simulink model "ATOM_parking_chain"  (R2026a)
settings: Solver=ode4  StopTime=100  FixedStep=0.01
StopFcn:
  | % Put every new figure in the same MATLAB Figures window as a docked tab.
  | set(groot, 'defaultFigureWindowStyle', 'docked');
  | 
  | if exist('costmap_active', 'var') && ...
  |         exist('vehicle', 'var') && ...
  |         exist('parking_path', 'var') && ...
  |         ~isempty(parking_path)
  | 
  |     plotPlan(costmap_active, vehicle, parking_path);
  | 
  | else
  | 
  |     warning('No valid parking path is available for plotting.');
  | 
  | end
  | 
  | PlotControllerReferences( ...
  |     out.controller_reference_log);
  | 
  | PlotControllerTracking( ...
  |     out.controller_tracking_log);
undefined symbols (not defined in the file): lateral, longitudinal, stanley, vehicle
(part 2 of 11)

== system ATOM_parking_chain/time_parameterization2 ==
  trajectory_in : Inport
  steer_rate_limit : Inport  Port=2
  Time parameterization : MATLAB Function  TreatAsAtomicUnit=on
  To Workspace : ToWorkspace  VariableName=time_parameterized_reference_log  SaveFormat=Timeseries  SampleTime=-1
  reference_out : Outport
  wires:
  trajectory_in/1 -> Time parameterization/1(trajectory_in)
  Time parameterization/1(reference_out) -> To Workspace/1, reference_out/1
  steer_rate_limit/1 -> Time parameterization/2(steer_rate_limit)

== system ATOM_parking_chain/Parking Scenario/Costmap generation: complex parking situation ==
  From Workspace1 : FromWorkspace  VariableName=veh
  MATLAB Function : MATLAB Function  TreatAsAtomicUnit=on
  costmap : Outport
  start_pose : Outport  Port=2
  goal_pose : Outport  Port=3
  wires:
  MATLAB Function/1(costmap) -> costmap/1
  From Workspace1/1 -> MATLAB Function/1(veh)
  MATLAB Function/2(start_pose) -> start_pose/1
  MATLAB Function/3(goal_pose) -> goal_pose/1

== system ATOM_parking_chain/Parking Scenario/Costmap generation: corridor occupancy grid ==
  From Workspace1 : FromWorkspace  VariableName=veh
  MATLAB Function : MATLAB Function  TreatAsAtomicUnit=on
  costmap : Outport
  start_pose : Outport  Port=2
  goal_pose : Outport  Port=3
  wires:
  MATLAB Function/1(costmap) -> costmap/1
  From Workspace1/1 -> MATLAB Function/1(veh)
  MATLAB Function/3(goal_pose) -> goal_pose/1
  MATLAB Function/2(start_pose) -> start_pose/1

== system ATOM_parking_chain/Parking Scenario/Costmap generation: empty occupancy grid ==
  From Workspace1 : FromWorkspace  VariableName=veh
  MATLAB Function : MATLAB Function  TreatAsAtomicUnit=on
  costmap : Outport
  start_pose : Outport  Port=2
  goal_pose : Outport  Port=3
  wires:
  MATLAB Function/1(costmap) -> costmap/1
  From Workspace1/1 -> MATLAB Function/1(veh)
  MATLAB Function/2(start_pose) -> start_pose/1
  MATLAB Function/3(goal_pose) -> goal_pose/1

== system ATOM_parking_chain/Parking Scenario/Costmap generation: obstacle ==
  From Workspace1 : FromWorkspace  VariableName=veh
  MATLAB Function : MATLAB Function  TreatAsAtomicUnit=on
  costmap : Outport
  start_pose : Outport  Port=2
  goal_pose : Outport  Port=3
  wires:
  MATLAB Function/1(costmap) -> costmap/1
  From Workspace1/1 -> MATLAB Function/1(veh)
  MATLAB Function/2(start_pose) -> start_pose/1
  MATLAB Function/3(goal_pose) -> goal_pose/1

== system ATOM_parking_chain/Parking Scenario/Costmap generation: obstacle1 ==
  From Workspace1 : FromWorkspace  VariableName=veh
  MATLAB Function : MATLAB Function  TreatAsAtomicUnit=on
  costmap : Outport
  start_pose : Outport  Port=2
  goal_pose : Outport  Port=3
  wires:
  MATLAB Function/1(costmap) -> costmap/1
  From Workspace1/1 -> MATLAB Function/1(veh)
  MATLAB Function/2(start_pose) -> start_pose/1
  MATLAB Function/3(goal_pose) -> goal_pose/1

== system ATOM_parking_chain/Parking Scenario/Costmap generation: obstacle2 ==
  From Workspace1 : FromWorkspace  VariableName=veh
  MATLAB Function : MATLAB Function  TreatAsAtomicUnit=on
  costmap : Outport
  start_pose : Outport  Port=2
  goal_pose : Outport  Port=3
  wires:
  MATLAB Function/1(costmap) -> costmap/1
  From Workspace1/1 -> MATLAB Function/1(veh)
  MATLAB Function/2(start_pose) -> start_pose/1
  MATLAB Function/3(goal_pose) -> goal_pose/1

== system ATOM_parking_chain/Parking Scenario/Costmap generation: parking scenario beside a lane ==
  From Workspace1 : FromWorkspace  VariableName=veh
  MATLAB Function : MATLAB Function  TreatAsAtomicUnit=on
  costmap : Outport
  start_pose : Outport  Port=2
  goal_pose : Outport  Port=3
  wires:
  MATLAB Function/1(costmap) -> costmap/1
  From Workspace1/1 -> MATLAB Function/1(veh)
  MATLAB Function/2(start_pose) -> start_pose/1
  MATLAB Function/3(goal_pose) -> goal_pose/1

== system ATOM_parking_chain/Parking Scenario/Costmap generation: perpendicular lot ==
  From Workspace1 : FromWorkspace  VariableName=veh
  Perpendicular Parking : MATLAB Function  TreatAsAtomicUnit=on
  costmap : Outport
  start_pose : Outport  Port=2
  goal_pose : Outport  Port=3
  wires:
  Perpendicular Parking/1(costmap) -> costmap/1
  From Workspace1/1 -> Perpendicular Parking/1(veh)
  Perpendicular Parking/2(start_pose) -> start_pose/1
  Perpendicular Parking/3(goal_pose) -> goal_pose/1

== system ATOM_parking_chain/Parking Scenario/freespace_planner ==
  costmap : Inport
  veh : Inport  Port=2
  goal_pose : Inport  Port=3
  start_pose : Inport  Port=4
  segment_request : Inport  Port=5
  Bus Creator3 : BusCreator  Inputs=3  OutDataTypeStr=Bus: PointBusN
  Bus Creator4 : BusCreator  Inputs=4  OutDataTypeStr=Bus: QuaternionBusN
  Bus Creator5 : BusCreator  Inputs=2  OutDataTypeStr=Bus: PoseBusN
      settings: InheritFromInputs=off
  Bus Creator6 : BusCreator  Inputs=7  OutDataTypeStr=Bus: TrajectoryDataBus
      settings: InheritFromInputs=off
  freespacePlanner : MATLAB Function  TreatAsAtomicUnit=on
  traj : Outport
  segment_count : Outport  Port=2
  wires:
  Bus Creator6/1 -> traj/1
  Bus Creator3/1 -> Bus Creator5/1
  freespacePlanner/13(rear_wheel_angle_rad) -> Bus Creator6/7
  Bus Creator5/1 -> Bus Creator6/1
  freespacePlanner/8(longitudinal_velocity_mps) -> Bus Creator6/2
  freespacePlanner/3(z) -> Bus Creator3/3
  freespacePlanner/4(qx) -> Bus Creator4/1
  freespacePlanner/9(lateral_velocity_mps) -> Bus Creator6/3
  freespacePlanner/10(acceleration_mps2) -> Bus Creator6/4
  freespacePlanner/5(qy) -> Bus Creator4/2
  freespacePlanner/1(x) -> Bus Creator3/1
  freespacePlanner/2(y) -> Bus Creator3/2
  freespacePlanner/7(qw) -> Bus Creator4/4
  freespacePlanner/6(qz) -> Bus Creator4/3
  freespacePlanner/12(front_wheel_angle_rad) -> Bus Creator6/6
  Bus Creator4/1 -> Bus Creator5/2
  freespacePlanner/11(heading_rate_rps) -> Bus Creator6/5
  costmap/1 -> freespacePlanner/4(costmap)
  start_pose/1 -> freespacePlanner/1(start_pose)
  goal_pose/1 -> freespacePlanner/2(goal_pose)
  veh/1 -> freespacePlanner/3(veh)
  segment_request/1 -> freespacePlanner/5(segment_request)
  freespacePlanner/14(segment_count) -> segment_count/1

== system ATOM_parking_chain/Parking Scenario1/Costmap generation: complex parking situation ==
  From Workspace1 : FromWorkspace  VariableName=veh
  MATLAB Function : MATLAB Function  TreatAsAtomicUnit=on
  costmap : Outport
  start_pose : Outport  Port=2
  goal_pose : Outport  Port=3
  wires:
  MATLAB Function/1(costmap) -> costmap/1
  From Workspace1/1 -> MATLAB Function/1(veh)
  MATLAB Function/2(start_pose) -> start_pose/1
  MATLAB Function/3(goal_pose) -> goal_pose/1

== system ATOM_parking_chain/Parking Scenario1/Costmap generation: corridor occupancy grid ==
  From Workspace1 : FromWorkspace  VariableName=veh
  MATLAB Function : MATLAB Function  TreatAsAtomicUnit=on
  costmap : Outport
  start_pose : Outport  Port=2
  goal_pose : Outport  Port=3
  wires:
  MATLAB Function/1(costmap) -> costmap/1
  From Workspace1/1 -> MATLAB Function/1(veh)
  MATLAB Function/3(goal_pose) -> goal_pose/1
  MATLAB Function/2(start_pose) -> start_pose/1

== system ATOM_parking_chain/Parking Scenario1/Costmap generation: empty occupancy grid ==
  From Workspace1 : FromWorkspace  VariableName=veh
  MATLAB Function : MATLAB Function  TreatAsAtomicUnit=on
  costmap : Outport
  start_pose : Outport  Port=2
  goal_pose : Outport  Port=3
  wires:
  MATLAB Function/1(costmap) -> costmap/1
  From Workspace1/1 -> MATLAB Function/1(veh)
  MATLAB Function/2(start_pose) -> start_pose/1
  MATLAB Function/3(goal_pose) -> goal_pose/1

== system ATOM_parking_chain/Parking Scenario1/Costmap generation: obstacle ==
  From Workspace1 : FromWorkspace  VariableName=veh
  MATLAB Function : MATLAB Function  TreatAsAtomicUnit=on
  costmap : Outport
  start_pose : Outport  Port=2
  goal_pose : Outport  Port=3
  wires:
  MATLAB Function/1(costmap) -> costmap/1
  From Workspace1/1 -> MATLAB Function/1(veh)
  MATLAB Function/2(start_pose) -> start_pose/1
  MATLAB Function/3(goal_pose) -> goal_pose/1

== system ATOM_parking_chain/Parking Scenario1/Costmap generation: obstacle1 ==
  From Workspace1 : FromWorkspace  VariableName=veh
  MATLAB Function : MATLAB Function  TreatAsAtomicUnit=on
  costmap : Outport
  start_pose : Outport  Port=2
  goal_pose : Outport  Port=3
  wires:
  MATLAB Function/1(costmap) -> costmap/1
  From Workspace1/1 -> MATLAB Function/1(veh)
  MATLAB Function/2(start_pose) -> start_pose/1
  MATLAB Function/3(goal_pose) -> goal_pose/1

== system ATOM_parking_chain/Parking Scenario1/Costmap generation: obstacle2 ==
  From Workspace1 : FromWorkspace  VariableName=veh
  MATLAB Function : MATLAB Function  TreatAsAtomicUnit=on
  costmap : Outport
  start_pose : Outport  Port=2
  goal_pose : Outport  Port=3
  wires:
  MATLAB Function/1(costmap) -> costmap/1
  From Workspace1/1 -> MATLAB Function/1(veh)
  MATLAB Function/2(start_pose) -> start_pose/1
  MATLAB Function/3(goal_pose) -> goal_pose/1

== system ATOM_parking_chain/Parking Scenario1/Costmap generation: parking scenario beside a lane ==
  From Workspace1 : FromWorkspace  VariableName=veh
  MATLAB Function : MATLAB Function  TreatAsAtomicUnit=on
  costmap : Outport
  start_pose : Outport  Port=2
  goal_pose : Outport  Port=3
  wires:
  MATLAB Function/1(costmap) -> costmap/1
  From Workspace1/1 -> MATLAB Function/1(veh)
  MATLAB Function/2(start_pose) -> start_pose/1
  MATLAB Function/3(goal_pose) -> goal_pose/1

== system ATOM_parking_chain/Parking Scenario1/Costmap generation: perpendicular lot ==
  From Workspace1 : FromWorkspace  VariableName=veh
  Perpendicular Parking : MATLAB Function  TreatAsAtomicUnit=on
  costmap : Outport
  start_pose : Outport  Port=2
  goal_pose : Outport  Port=3
  wires:
  Perpendicular Parking/1(costmap) -> costmap/1
  From Workspace1/1 -> Perpendicular Parking/1(veh)
  Perpendicular Parking/2(start_pose) -> start_pose/1
  Perpendicular Parking/3(goal_pose) -> goal_pose/1

== system ATOM_parking_chain/Parking Scenario1/freespace_planner ==
  costmap : Inport
  veh : Inport  Port=2
  goal_pose : Inport  Port=3
  start_pose : Inport  Port=4
  segment_request : Inport  Port=5
  Bus Creator3 : BusCreator  Inputs=3  OutDataTypeStr=Bus: PointBusN
  Bus Creator4 : BusCreator  Inputs=4  OutDataTypeStr=Bus: QuaternionBusN
  Bus Creator5 : BusCreator  Inputs=2  OutDataTypeStr=Bus: PoseBusN
      settings: InheritFromInputs=off
  Bus Creator6 : BusCreator  Inputs=7  OutDataTypeStr=Bus: TrajectoryDataBus
      settings: InheritFromInputs=off
  freespacePlanner : MATLAB Function  TreatAsAtomicUnit=on
  traj : Outport
  segment_count : Outport  Port=2
  wires:
  Bus Creator6/1 -> traj/1
  Bus Creator3/1 -> Bus Creator5/1
  freespacePlanner/13(rear_wheel_angle_rad) -> Bus Creator6/7
  Bus Creator5/1 -> Bus Creator6/1
  freespacePlanner/8(longitudinal_velocity_mps) -> Bus Creator6/2
  freespacePlanner/3(z) -> Bus Creator3/3
  freespacePlanner/4(qx) -> Bus Creator4/1
  freespacePlanner/9(lateral_velocity_mps) -> Bus Creator6/3
  freespacePlanner/10(acceleration_mps2) -> Bus Creator6/4
  freespacePlanner/5(qy) -> Bus Creator4/2
  freespacePlanner/1(x) -> Bus Creator3/1
  freespacePlanner/2(y) -> Bus Creator3/2
  freespacePlanner/7(qw) -> Bus Creator4/4
  freespacePlanner/6(qz) -> Bus Creator4/3
  freespacePlanner/12(front_wheel_angle_rad) -> Bus Creator6/6
  Bus Creator4/1 -> Bus Creator5/2
  freespacePlanner/11(heading_rate_rps) -> Bus Creator6/5
  costmap/1 -> freespacePlanner/4(costmap)
  start_pose/1 -> freespacePlanner/1(start_pose)
  goal_pose/1 -> freespacePlanner/2(goal_pose)
  veh/1 -> freespacePlanner/3(veh)
  segment_request/1 -> freespacePlanner/5(segment_request)
  freespacePlanner/14(segment_count) -> segment_count/1

== system ATOM_parking_chain/Parking Scenario2/Costmap generation: complex parking situation ==
  From Workspace1 : FromWorkspace  VariableName=veh
  MATLAB Function : MATLAB Function  TreatAsAtomicUnit=on
  costmap : Outport
  start_pose : Outport  Port=2
  goal_pose : Outport  Port=3
  wires:
  MATLAB Function/1(costmap) -> costmap/1
  From Workspace1/1 -> MATLAB Function/1(veh)
  MATLAB Function/2(start_pose) -> start_pose/1
  MATLAB Function/3(goal_pose) -> goal_pose/1

== system ATOM_parking_chain/Parking Scenario2/Costmap generation: corridor occupancy grid ==
  From Workspace1 : FromWorkspace  VariableName=veh
  MATLAB Function : MATLAB Function  TreatAsAtomicUnit=on
  costmap : Outport
  start_pose : Outport  Port=2
  goal_pose : Outport  Port=3
  wires:
  MATLAB Function/1(costmap) -> costmap/1
  From Workspace1/1 -> MATLAB Function/1(veh)
  MATLAB Function/3(goal_pose) -> goal_pose/1
  MATLAB Function/2(start_pose) -> start_pose/1

== system ATOM_parking_chain/Parking Scenario2/Costmap generation: empty occupancy grid ==
  From Workspace1 : FromWorkspace  VariableName=veh
  MATLAB Function : MATLAB Function  TreatAsAtomicUnit=on
  costmap : Outport
  start_pose : Outport  Port=2
  goal_pose : Outport  Port=3
  wires:
  MATLAB Function/1(costmap) -> costmap/1
  From Workspace1/1 -> MATLAB Function/1(veh)
  MATLAB Function/2(start_pose) -> start_pose/1
  MATLAB Function/3(goal_pose) -> goal_pose/1

== system ATOM_parking_chain/Parking Scenario2/Costmap generation: obstacle ==
  From Workspace1 : FromWorkspace  VariableName=veh
  MATLAB Function : MATLAB Function  TreatAsAtomicUnit=on
  costmap : Outport
  start_pose : Outport  Port=2
  goal_pose : Outport  Port=3
  wires:
  MATLAB Function/1(costmap) -> costmap/1
  From Workspace1/1 -> MATLAB Function/1(veh)
  MATLAB Function/2(start_pose) -> start_pose/1
  MATLAB Function/3(goal_pose) -> goal_pose/1

== system ATOM_parking_chain/Parking Scenario2/Costmap generation: obstacle1 ==
  From Workspace1 : FromWorkspace  VariableName=veh
  MATLAB Function : MATLAB Function  TreatAsAtomicUnit=on
  costmap : Outport
  start_pose : Outport  Port=2
  goal_pose : Outport  Port=3
  wires:
  MATLAB Function/1(costmap) -> costmap/1
  From Workspace1/1 -> MATLAB Function/1(veh)
  MATLAB Function/2(start_pose) -> start_pose/1
  MATLAB Function/3(goal_pose) -> goal_pose/1

== system ATOM_parking_chain/Parking Scenario2/Costmap generation: obstacle2 ==
  From Workspace1 : FromWorkspace  VariableName=veh
  MATLAB Function : MATLAB Function  TreatAsAtomicUnit=on
  costmap : Outport
  start_pose : Outport  Port=2
  goal_pose : Outport  Port=3
  wires:
  MATLAB Function/1(costmap) -> costmap/1
  From Workspace1/1 -> MATLAB Function/1(veh)
  MATLAB Function/2(start_pose) -> start_pose/1
  MATLAB Function/3(goal_pose) -> goal_pose/1

== system ATOM_parking_chain/Parking Scenario2/Costmap generation: parking scenario beside a lane ==
  From Workspace1 : FromWorkspace  VariableName=veh
  MATLAB Function : MATLAB Function  TreatAsAtomicUnit=on
  costmap : Outport
  start_pose : Outport  Port=2
  goal_pose : Outport  Port=3
  wires:
  MATLAB Function/1(costmap) -> costmap/1
  From Workspace1/1 -> MATLAB Function/1(veh)
  MATLAB Function/2(start_pose) -> start_pose/1
  MATLAB Function/3(goal_pose) -> goal_pose/1

== system ATOM_parking_chain/Parking Scenario2/Costmap generation: perpendicular lot ==
  From Workspace1 : FromWorkspace  VariableName=veh
  Perpendicular Parking : MATLAB Function  TreatAsAtomicUnit=on
  costmap : Outport
  start_pose : Outport  Port=2
  goal_pose : Outport  Port=3
  wires:
  Perpendicular Parking/1(costmap) -> costmap/1
  From Workspace1/1 -> Perpendicular Parking/1(veh)
  Perpendicular Parking/2(start_pose) -> start_pose/1
  Perpendicular Parking/3(goal_pose) -> goal_pose/1

== system ATOM_parking_chain/Parking Scenario2/freespace_planner ==
  costmap : Inport
  veh : Inport  Port=2
  goal_pose : Inport  Port=3
  start_pose : Inport  Port=4
  segment_request : Inport  Port=5
  Bus Creator3 : BusCreator  Inputs=3  OutDataTypeStr=Bus: PointBusN
  Bus Creator4 : BusCreator  Inputs=4  OutDataTypeStr=Bus: QuaternionBusN
  Bus Creator5 : BusCreator  Inputs=2  OutDataTypeStr=Bus: PoseBusN
      settings: InheritFromInputs=off
  Bus Creator6 : BusCreator  Inputs=7  OutDataTypeStr=Bus: TrajectoryDataBus
      settings: InheritFromInputs=off
  freespacePlanner : MATLAB Function  TreatAsAtomicUnit=on
  traj : Outport
  segment_count : Outport  Port=2
  wires:
  Bus Creator6/1 -> traj/1
  Bus Creator3/1 -> Bus Creator5/1
  freespacePlanner/13(rear_wheel_angle_rad) -> Bus Creator6/7
  Bus Creator5/1 -> Bus Creator6/1
  freespacePlanner/8(longitudinal_velocity_mps) -> Bus Creator6/2
  freespacePlanner/3(z) -> Bus Creator3/3
  freespacePlanner/4(qx) -> Bus Creator4/1
  freespacePlanner/9(lateral_velocity_mps) -> Bus Creator6/3
  freespacePlanner/10(acceleration_mps2) -> Bus Creator6/4
  freespacePlanner/5(qy) -> Bus Creator4/2
  freespacePlanner/1(x) -> Bus Creator3/1
  freespacePlanner/2(y) -> Bus Creator3/2
  freespacePlanner/7(qw) -> Bus Creator4/4
  freespacePlanner/6(qz) -> Bus Creator4/3
  freespacePlanner/12(front_wheel_angle_rad) -> Bus Creator6/6
  Bus Creator4/1 -> Bus Creator5/2
  freespacePlanner/11(heading_rate_rps) -> Bus Creator6/5
  costmap/1 -> freespacePlanner/4(costmap)
  start_pose/1 -> freespacePlanner/1(start_pose)
  goal_pose/1 -> freespacePlanner/2(goal_pose)
  veh/1 -> freespacePlanner/3(veh)
  segment_request/1 -> freespacePlanner/5(segment_request)
  freespacePlanner/14(segment_count) -> segment_count/1

== system ATOM_parking_chain/Plot vehicle1/SetStanleyTrajectory ==
  ref_traj : Inport
  ego_pose : Inport  Port=2
  Constant1 : Constant  Value=stanley.traj_resample_dist
  Resample Trajectory : MATLAB Function  TreatAsAtomicUnit=on
  calcLongOffsetToSegment : MATLAB Function  TreatAsAtomicUnit=on
  default : Constant  Value=3
  default1 : Constant  Value=pi/2
  findFirstNearestSegmentIndexWithSoftConstraints : MATLAB Function  TreatAsAtomicUnit=on
  trajectory_out : Outport
  wires:
  ref_traj/1 -> Resample Trajectory/1(trajectory_in), calcLongOffsetToSegment/3(trajectory), findFirstNearestSegmentIndexWithSoftConstraints/1(trajectory)
  Constant1/1 -> Resample Trajectory/2(resample_interval_dist)
  calcLongOffsetToSegment/1(ego_offset_to_segment) -> Resample Trajectory/4(ego_offset_to_segment)
  ego_pose/1 -> findFirstNearestSegmentIndexWithSoftConstraints/4(pose), calcLongOffsetToSegment/2(ego_pose)
  findFirstNearestSegmentIndexWithSoftConstraints/1(nearest_seg_idx) -> calcLongOffsetToSegment/1(seg_idx), Resample Trajectory/3(nearest_seg_idx)
  default/1 -> findFirstNearestSegmentIndexWithSoftConstraints/2(dist_threshold)
  default1/1 -> findFirstNearestSegmentIndexWithSoftConstraints/3(yaw_threshold)
  Resample Trajectory/1(trajectory_out) -> trajectory_out/1

== system ATOM_parking_chain/Plot vehicle2/SetStanleyTrajectory ==
  ref_traj : Inport
  ego_pose : Inport  Port=2
  Constant1 : Constant  Value=stanley.traj_resample_dist
  Resample Trajectory : MATLAB Function  TreatAsAtomicUnit=on
  calcLongOffsetToSegment : MATLAB Function  TreatAsAtomicUnit=on
  default : Constant  Value=3
  default1 : Constant  Value=pi/2
  findFirstNearestSegmentIndexWithSoftConstraints : MATLAB Function  TreatAsAtomicUnit=on
  trajectory_out : Outport
  wires:
  ref_traj/1 -> Resample Trajectory/1(trajectory_in), calcLongOffsetToSegment/3(trajectory), findFirstNearestSegmentIndexWithSoftConstraints/1(trajectory)
  Constant1/1 -> Resample Trajectory/2(resample_interval_dist)
  calcLongOffsetToSegment/1(ego_offset_to_segment) -> Resample Trajectory/4(ego_offset_to_segment)
  ego_pose/1 -> findFirstNearestSegmentIndexWithSoftConstraints/4(pose), calcLongOffsetToSegment/2(ego_pose)
  findFirstNearestSegmentIndexWithSoftConstraints/1(nearest_seg_idx) -> calcLongOffsetToSegment/1(seg_idx), Resample Trajectory/3(nearest_seg_idx)
  default/1 -> findFirstNearestSegmentIndexWithSoftConstraints/2(dist_threshold)
  default1/1 -> findFirstNearestSegmentIndexWithSoftConstraints/3(yaw_threshold)
  Resample Trajectory/1(trajectory_out) -> trajectory_out/1

== system ATOM_parking_chain/Plot vehicle3/SetStanleyTrajectory ==
  ref_traj : Inport
  ego_pose : Inport  Port=2
  Constant1 : Constant  Value=stanley.traj_resample_dist
  Resample Trajectory : MATLAB Function  TreatAsAtomicUnit=on
  calcLongOffsetToSegment : MATLAB Function  TreatAsAtomicUnit=on
  default : Constant  Value=3
  default1 : Constant  Value=pi/2
  findFirstNearestSegmentIndexWithSoftConstraints : MATLAB Function  TreatAsAtomicUnit=on
  trajectory_out : Outport
  wires:
  ref_traj/1 -> Resample Trajectory/1(trajectory_in), calcLongOffsetToSegment/3(trajectory), findFirstNearestSegmentIndexWithSoftConstraints/1(trajectory)
  Constant1/1 -> Resample Trajectory/2(resample_interval_dist)
  calcLongOffsetToSegment/1(ego_offset_to_segment) -> Resample Trajectory/4(ego_offset_to_segment)
  ego_pose/1 -> findFirstNearestSegmentIndexWithSoftConstraints/4(pose), calcLongOffsetToSegment/2(ego_pose)
  findFirstNearestSegmentIndexWithSoftConstraints/1(nearest_seg_idx) -> calcLongOffsetToSegment/1(seg_idx), Resample Trajectory/3(nearest_seg_idx)
  default/1 -> findFirstNearestSegmentIndexWithSoftConstraints/2(dist_threshold)
  default1/1 -> findFirstNearestSegmentIndexWithSoftConstraints/3(yaw_threshold)
  Resample Trajectory/1(trajectory_out) -> trajectory_out/1

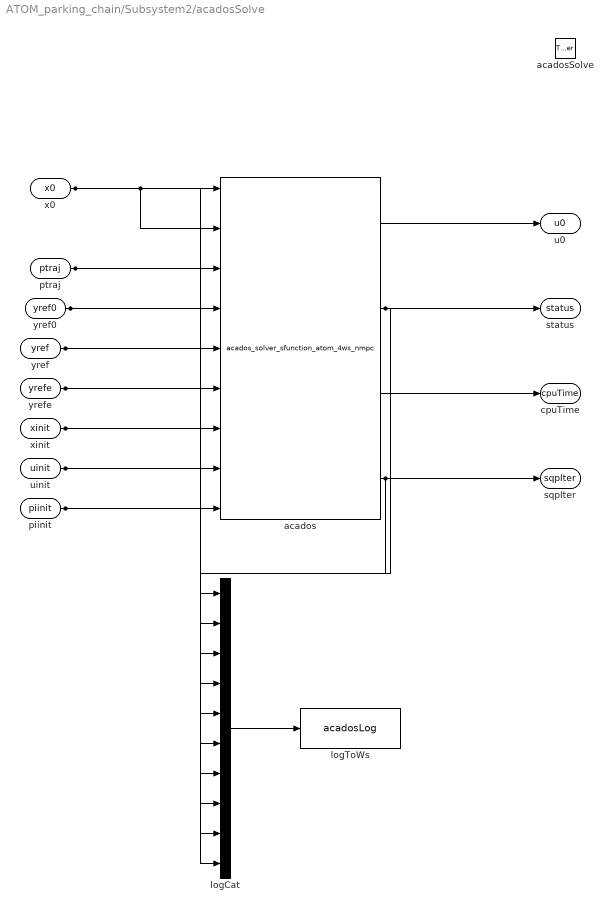
== system ATOM_parking_chain/Subsystem2/acadosSolve ==
  acadosSolve : TriggerPort  TriggerType=function-call  IsSimulinkFunction=on  FunctionName=acadosSolve  FunctionVisibility=scoped  VariantControl=(inherit)
  acados : S-Function  FunctionName=acados_solver_sfunction_atom_4ws_nmpc  SFunctionDeploymentMode=off  EnableBusSupport=off
  logCat : Concatenate  NumInputs=10
  logToWs : ToWorkspace  VariableName=acadosLog  SaveFormat=Structure With Time  SampleTime=-1
  x0 : ArgIn  DisableCoverage=on  PortDimensions=[9 1]  ArgumentName=x0
  ptraj : ArgIn  Port=2  PortDimensions=[272 1]  ArgumentName=ptraj
  yref0 : ArgIn  Port=3  PortDimensions=[7 1]  ArgumentName=yref0
  yref : ArgIn  Port=4  PortDimensions=[98 1]  ArgumentName=yref
  yrefe : ArgIn  Port=5  PortDimensions=[5 1]  ArgumentName=yrefe
  xinit : ArgIn  Port=6  PortDimensions=[144 1]  ArgumentName=xinit
  uinit : ArgIn  Port=7  PortDimensions=[30 1]  ArgumentName=uinit
  piinit : ArgIn  Port=8  PortDimensions=[135 1]  ArgumentName=piinit
  u0 : ArgOut  DisableCoverage=on  PortDimensions=[2 1]  ArgumentName=u0
  status : ArgOut  Port=2  ArgumentName=status
  cpuTime : ArgOut  Port=3  ArgumentName=cpuTime
  sqpIter : ArgOut  Port=4  ArgumentName=sqpIter
  wires:
  x0/1 -> acados/1, acados/2, logCat/1
  ptraj/1 -> acados/3, logCat/2
  yref0/1 -> acados/4, logCat/3
  yref/1 -> acados/5, logCat/4
  yrefe/1 -> acados/6, logCat/5
  xinit/1 -> acados/7, logCat/6
  uinit/1 -> acados/8, logCat/7
  piinit/1 -> acados/9, logCat/8
  acados/1 -> u0/1
  acados/2 -> status/1, logCat/9
  acados/3 -> cpuTime/1
  acados/4 -> sqpIter/1, logCat/10
  logCat/1 -> logToWs/1

== system ATOM_parking_chain/Vehicle_Model/Vehicle Dynamics ==
  command : Inport
  rear_steer_command : Inport  Port=2
  From Workspace : FromWorkspace  VariableName=veh
  MATLAB Function : MATLAB Function  TreatAsAtomicUnit=on
  state integrator : Subsystem
  IntState : Outport
  wires:
  command/1 -> MATLAB Function/2(command)
  MATLAB Function/1(d_state) -> state integrator/1(d_state)  "d_state"
  state integrator/1(state) -> MATLAB Function/1(state), IntState/1
  From Workspace/1 -> MATLAB Function/3(veh)
  rear_steer_command/1 -> MATLAB Function/4(rear_steering_command)

== system ATOM_parking_chain/Vehicle_Model/Vehicle internal state ==
  IntState : Inport
  Bus Selector : BusSelector  OutputSignals=x,y,yaw,vx,steer_front,steer_rear,acc
  Scope{,1..6} (7 alike) : Scope
      Scope settings: ActiveDisplayYMinimum=-1  ActiveDisplayYMaximum=1
      Scope1 settings: ActiveDisplayYMinimum=-1  ActiveDisplayYMaximum=1
      Scope2 settings: ActiveDisplayYMinimum=-1  ActiveDisplayYMaximum=1  DataLoggingVariableName=ScopeData2
      Scope3 settings: ActiveDisplayYMinimum=-1  ActiveDisplayYMaximum=1  DataLoggingVariableName=ScopeData3
      Scope4 settings: ActiveDisplayYMinimum=-1  ActiveDisplayYMaximum=1  DataLoggingVariableName=ScopeData4
      Scope5 settings: ActiveDisplayYMinimum=-1  ActiveDisplayYMaximum=1  DataLoggingVariableName=ScopeData5
      Scope6 settings: ActiveDisplayYMinimum=-1  ActiveDisplayYMaximum=1  DataLoggingVariableName=ScopeData6
  steer_front : Outport
  steer_rear : Outport  Port=2
  wires:
  Bus Selector/2 -> Scope1/1  "<y>"
  Bus Selector/4 -> Scope3/1  "<vx>"
  Bus Selector/1 -> Scope/1  "<x>"
  Bus Selector/3 -> Scope2/1  "<yaw>"
  Bus Selector/7 -> Scope6/1  "<acc>"
  Bus Selector/5 -> steer_front/1, Scope4/1  "<steer_front>"
  Bus Selector/6 -> steer_rear/1, Scope5/1  "<steer_rear>"
  IntState/1 -> Bus Selector/1

== system ATOM_parking_chain/Vehicle_Model1/Vehicle Dynamics ==
  command : Inport
  rear_steer_command : Inport  Port=2
  From Workspace : FromWorkspace  VariableName=veh
  MATLAB Function : MATLAB Function  TreatAsAtomicUnit=on
  state integrator : Subsystem
  IntState : Outport
  wires:
  command/1 -> MATLAB Function/2(command)
  MATLAB Function/1(d_state) -> state integrator/1(d_state)  "d_state"
  state integrator/1(state) -> MATLAB Function/1(state), IntState/1
  From Workspace/1 -> MATLAB Function/3(veh)
  rear_steer_command/1 -> MATLAB Function/4(rear_steering_command)

== system ATOM_parking_chain/Vehicle_Model1/Vehicle internal state ==
  IntState : Inport
  Bus Selector : BusSelector  OutputSignals=x,y,yaw,vx,steer_front,steer_rear,acc
  Scope{,1..6} (7 alike) : Scope
      Scope settings: ActiveDisplayYMinimum=-1  ActiveDisplayYMaximum=1
      Scope1 settings: ActiveDisplayYMinimum=-1  ActiveDisplayYMaximum=1
      Scope2 settings: ActiveDisplayYMinimum=-1  ActiveDisplayYMaximum=1  DataLoggingVariableName=ScopeData2
      Scope3 settings: ActiveDisplayYMinimum=-1  ActiveDisplayYMaximum=1  DataLoggingVariableName=ScopeData3
      Scope4 settings: ActiveDisplayYMinimum=-1  ActiveDisplayYMaximum=1  DataLoggingVariableName=ScopeData4
      Scope5 settings: ActiveDisplayYMinimum=-1  ActiveDisplayYMaximum=1  DataLoggingVariableName=ScopeData5
      Scope6 settings: ActiveDisplayYMinimum=-1  ActiveDisplayYMaximum=1  DataLoggingVariableName=ScopeData6
  steer_front : Outport
  steer_rear : Outport  Port=2
  wires:
  Bus Selector/2 -> Scope1/1  "<y>"
  Bus Selector/4 -> Scope3/1  "<vx>"
  Bus Selector/1 -> Scope/1  "<x>"
  Bus Selector/3 -> Scope2/1  "<yaw>"
  Bus Selector/7 -> Scope6/1  "<acc>"
  Bus Selector/5 -> steer_front/1, Scope4/1  "<steer_front>"
  Bus Selector/6 -> steer_rear/1, Scope5/1  "<steer_rear>"
  IntState/1 -> Bus Selector/1

== system ATOM_parking_chain/Vehicle_Model2/Vehicle Dynamics ==
  command : Inport
  rear_steer_command : Inport  Port=2
  From Workspace : FromWorkspace  VariableName=veh
  MATLAB Function : MATLAB Function  TreatAsAtomicUnit=on
  state integrator : Subsystem
  IntState : Outport
  wires:
  command/1 -> MATLAB Function/2(command)
  MATLAB Function/1(d_state) -> state integrator/1(d_state)  "d_state"
  state integrator/1(state) -> MATLAB Function/1(state), IntState/1
  From Workspace/1 -> MATLAB Function/3(veh)
  rear_steer_command/1 -> MATLAB Function/4(rear_steering_command)

== system ATOM_parking_chain/Vehicle_Model2/Vehicle internal state ==
  IntState : Inport
  Bus Selector : BusSelector  OutputSignals=x,y,yaw,vx,steer_front,steer_rear,acc
  Scope{,1..6} (7 alike) : Scope
      Scope settings: ActiveDisplayYMinimum=-1  ActiveDisplayYMaximum=1
      Scope1 settings: ActiveDisplayYMinimum=-1  ActiveDisplayYMaximum=1
      Scope2 settings: ActiveDisplayYMinimum=-1  ActiveDisplayYMaximum=1  DataLoggingVariableName=ScopeData2
      Scope3 settings: ActiveDisplayYMinimum=-1  ActiveDisplayYMaximum=1  DataLoggingVariableName=ScopeData3
      Scope4 settings: ActiveDisplayYMinimum=-1  ActiveDisplayYMaximum=1  DataLoggingVariableName=ScopeData4
      Scope5 settings: ActiveDisplayYMinimum=-1  ActiveDisplayYMaximum=1  DataLoggingVariableName=ScopeData5
      Scope6 settings: ActiveDisplayYMinimum=-1  ActiveDisplayYMaximum=1  DataLoggingVariableName=ScopeData6
  steer_front : Outport
  steer_rear : Outport  Port=2
  wires:
  Bus Selector/2 -> Scope1/1  "<y>"
  Bus Selector/4 -> Scope3/1  "<vx>"
  Bus Selector/1 -> Scope/1  "<x>"
  Bus Selector/3 -> Scope2/1  "<yaw>"
  Bus Selector/7 -> Scope6/1  "<acc>"
  Bus Selector/5 -> steer_front/1, Scope4/1  "<steer_front>"
  Bus Selector/6 -> steer_rear/1, Scope5/1  "<steer_rear>"
  IntState/1 -> Bus Selector/1

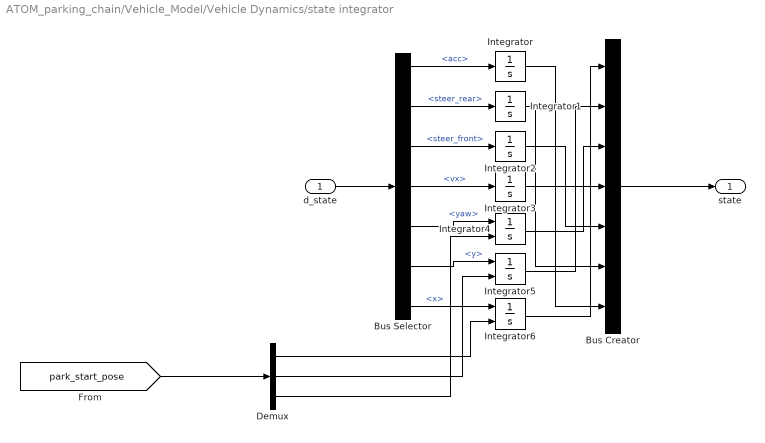
== system ATOM_parking_chain/Vehicle_Model/Vehicle Dynamics/state integrator ==
  d_state : Inport
  Bus Creator : BusCreator  Inputs=7  OutDataTypeStr=Bus: VehicleInternalStateBus
      settings: InheritFromInputs=off
  Bus Selector : BusSelector  OutputSignals=acc,steer_rear,steer_front,vx,yaw,y,x
  Demux : Demux  Outputs=3
  Integrator{,1..3} (4 alike) : Integrator
  Integrator4 : Integrator  InitialConditionSource=external
  Integrator5 : Integrator  InitialConditionSource=external
  Integrator6 : Integrator  InitialConditionSource=external  InitialCondition=-2
  state : Outport
  wires:
  Integrator4/1 -> Bus Creator/3
  Integrator3/1 -> Bus Creator/4
  Integrator6/1 -> Bus Creator/1
  Bus Selector/4 -> Integrator3/1  "<vx>"
  Integrator1/1 -> Bus Creator/6
  Bus Creator/1 -> state/1
  Bus Selector/6 -> Integrator5/1  "<y>"
  Bus Selector/2 -> Integrator1/1  "<steer_rear>"
  Integrator5/1 -> Bus Creator/2
  Bus Selector/7 -> Integrator6/1  "<x>"
  Bus Selector/3 -> Integrator2/1  "<steer_front>"
  Bus Selector/1 -> Integrator/1  "<acc>"
  Integrator/1 -> Bus Creator/7
  Bus Selector/5 -> Integrator4/1  "<yaw>"
  d_state/1 -> Bus Selector/1
  Integrator2/1 -> Bus Creator/5
  [park_start_pose] -> Demux/1
  Demux/1 -> Integrator6/2
  Demux/2 -> Integrator5/2
  Demux/3 -> Integrator4/2

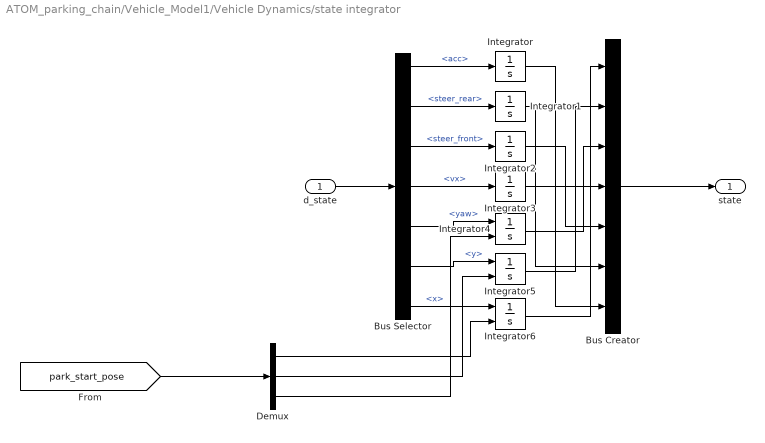
== system ATOM_parking_chain/Vehicle_Model1/Vehicle Dynamics/state integrator ==
  d_state : Inport
  Bus Creator : BusCreator  Inputs=7  OutDataTypeStr=Bus: VehicleInternalStateBus
      settings: InheritFromInputs=off
  Bus Selector : BusSelector  OutputSignals=acc,steer_rear,steer_front,vx,yaw,y,x
  Demux : Demux  Outputs=3
  Integrator{,1..3} (4 alike) : Integrator
  Integrator4 : Integrator  InitialConditionSource=external
  Integrator5 : Integrator  InitialConditionSource=external
  Integrator6 : Integrator  InitialConditionSource=external  InitialCondition=-2
  state : Outport
  wires:
  Integrator4/1 -> Bus Creator/3
  Integrator3/1 -> Bus Creator/4
  Integrator6/1 -> Bus Creator/1
  Bus Selector/4 -> Integrator3/1  "<vx>"
  Integrator1/1 -> Bus Creator/6
  Bus Creator/1 -> state/1
  Bus Selector/6 -> Integrator5/1  "<y>"
  Bus Selector/2 -> Integrator1/1  "<steer_rear>"
  Integrator5/1 -> Bus Creator/2
  Bus Selector/7 -> Integrator6/1  "<x>"
  Bus Selector/3 -> Integrator2/1  "<steer_front>"
  Bus Selector/1 -> Integrator/1  "<acc>"
  Integrator/1 -> Bus Creator/7
  Bus Selector/5 -> Integrator4/1  "<yaw>"
  d_state/1 -> Bus Selector/1
  Integrator2/1 -> Bus Creator/5
  [park_start_pose] -> Demux/1
  Demux/1 -> Integrator6/2
  Demux/2 -> Integrator5/2
  Demux/3 -> Integrator4/2

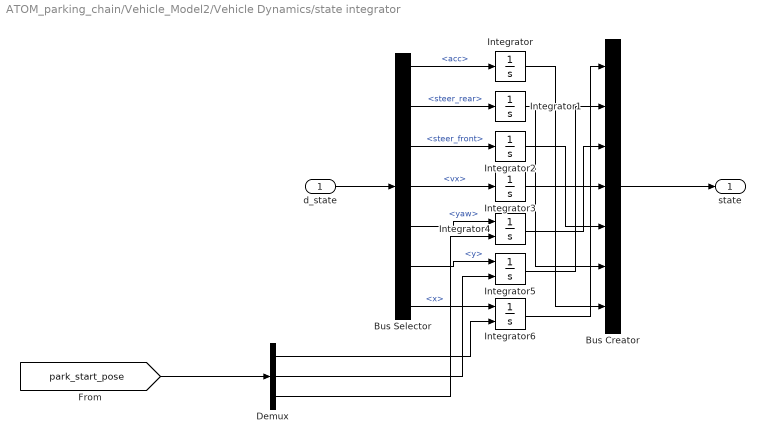
== system ATOM_parking_chain/Vehicle_Model2/Vehicle Dynamics/state integrator ==
  d_state : Inport
  Bus Creator : BusCreator  Inputs=7  OutDataTypeStr=Bus: VehicleInternalStateBus
      settings: InheritFromInputs=off
  Bus Selector : BusSelector  OutputSignals=acc,steer_rear,steer_front,vx,yaw,y,x
  Demux : Demux  Outputs=3
  Integrator{,1..3} (4 alike) : Integrator
  Integrator4 : Integrator  InitialConditionSource=external
  Integrator5 : Integrator  InitialConditionSource=external
  Integrator6 : Integrator  InitialConditionSource=external  InitialCondition=-2
  state : Outport
  wires:
  Integrator4/1 -> Bus Creator/3
  Integrator3/1 -> Bus Creator/4
  Integrator6/1 -> Bus Creator/1
  Bus Selector/4 -> Integrator3/1  "<vx>"
  Integrator1/1 -> Bus Creator/6
  Bus Creator/1 -> state/1
  Bus Selector/6 -> Integrator5/1  "<y>"
  Bus Selector/2 -> Integrator1/1  "<steer_rear>"
  Integrator5/1 -> Bus Creator/2
  Bus Selector/7 -> Integrator6/1  "<x>"
  Bus Selector/3 -> Integrator2/1  "<steer_front>"
  Bus Selector/1 -> Integrator/1  "<acc>"
  Integrator/1 -> Bus Creator/7
  Bus Selector/5 -> Integrator4/1  "<yaw>"
  d_state/1 -> Bus Selector/1
  Integrator2/1 -> Bus Creator/5
  [park_start_pose] -> Demux/1
  Demux/1 -> Integrator6/2
  Demux/2 -> Integrator5/2
  Demux/3 -> Integrator4/2

== matlab function ATOM_parking_chain/Parking Scenario1/Costmap generation: empty occupancy grid/MATLAB Function ==
  data: veh input; costmap output Bus: OccupancyGridBus; start_pose output; goal_pose output
function [costmap, start_pose, goal_pose] = costmapEmptyLot(veh) %#ok<INUSD>
%COSTMAPEMPTYLOT  Empty lot - no objects layer. The reference case:
% whatever the planner does here is forced by the turning radius alone,
% not by obstacles.
%
% veh is unused (no parked cars to size) but kept so all costmap blocks
% have identical ports and can be rewired freely.

persistent occ

res = 0.3;   W = 234;   H = 234;
origin_x = -(W/2)*res;
origin_y = -(H/2)*res;

if isempty(occ)
    [IX, IY] = meshgrid(0:W-1, 0:H-1);
    X = origin_x + IX*res;
    Y = origin_y + IY*res;

    lot_x = [-15  15  15 -15];
    lot_y = [-12 -12  12  12];
    occ = ones(H,W);
    occ(inpolygon(X, Y, lot_x, lot_y)) = 0;
end

start_pose = [-8, 0, 0];
goal_pose  = [ 0, 5, pi/2];

costmap.info.resolution           = res;
costmap.info.width                = uint32(W);
costmap.info.height               = uint32(H);
costmap.info.origin.position.x    = origin_x;
costmap.info.origin.position.y    = origin_y;
costmap.info.origin.position.z    = 0;
costmap.info.origin.orientation.x = 0;
costmap.info.origin.orientation.y = 0;
costmap.info.origin.orientation.z = 0;
costmap.info.origin.orientation.w = 1;
costmap.data                      = int8(occ*100);
end

== matlab function ATOM_parking_chain/Parking Scenario1/Costmap generation: obstacle/MATLAB Function ==
  settings: updateMethod=DISCRETE
  data: veh input; costmap output Bus: OccupancyGridBus; start_pose output; goal_pose output
function [costmap, start_pose, goal_pose] = costmapSingleObstacle(veh) %#ok<INUSD>
%COSTMAPSINGLEOBSTACLE  Open area with one obstacle blocking the direct route.
% Paste this function into the connected costmap MATLAB Function block.
% Poses refer to the rear-axle centre; headings are in radians.
% Keep the vehicle input so the existing Simulink connections still match.

% Fixed dimensions match the existing OccupancyGrid bus.
res = 0.2;
W = 234;
H = 234;
origin_x = -(W/2)*res;
origin_y = -(H/2)*res;

% Editable scene dimensions [m].
area_x_min = -14;
area_x_max =  14;
area_y_min =  -8;
area_y_max =   8;

obstacle_center_x = 0;
obstacle_center_y = 0;
obstacle_length = 3;  % Along x.
obstacle_width  = 5;  % Along y.

start_pose = [-8, 0, 0];
goal_pose  = [ 8, 0, 0];

% Rebuild each call so changes cannot leave an old persistent map active.
[IX, IY] = meshgrid(0:W-1, 0:H-1);
X = origin_x + IX*res;
Y = origin_y + IY*res;

% Outside the open area is occupied; inside is free.
occupied = ~(X >= area_x_min & X <= area_x_max & ...
             Y >= area_y_min & Y <= area_y_max);

% The physical obstacle is added without extra inflation. collisionCheck
% already includes the planner's vehicle-shape margin.
obstacle = abs(X-obstacle_center_x) <= obstacle_length/2 & ...
           abs(Y-obstacle_center_y) <= obstacle_width/2;
occupied = occupied | obstacle;

costmap.info.resolution = res;
costmap.info.width  = uint32(W);
costmap.info.height = uint32(H);

costmap.info.origin.position.x = origin_x;
costmap.info.origin.position.y = origin_y;
costmap.info.origin.position.z = 0;
costmap.info.origin.orientation.x = 0;
costmap.info.origin.orientation.y = 0;
costmap.info.origin.orientation.z = 0;
costmap.info.origin.orientation.w = 1;

% Preserve the existing H-by-W int8 bus payload: free=0, occupied=100.
costmap.data = int8(occupied) .* int8(100);
end

== matlab function ATOM_parking_chain/Parking Scenario1/Costmap generation: obstacle1/MATLAB Function ==
  settings: updateMethod=DISCRETE
  data: costmap output Bus: OccupancyGridBus; start_pose output; goal_pose output; veh input
function [costmap, start_pose, goal_pose] = costmapOffsetDock(veh)
%COSTMAPOFFSETDOCK  A short, angled parking bay beside a narrow aisle.
% Paste into a duplicate of an existing costmap MATLAB Function block.
% Inputs/outputs and the 234-by-234 int8 payload match the current model.
% Poses refer to the rear-axle centre; headings are in radians.

%% Map and scene dimensions [m]
res = 0.20;
W = 234;
H = 234;
origin_x = -(W/2)*res;
origin_y = -(H/2)*res;

aisle_width = 3.20;
aisle_x_min = -8.9;
aisle_x_max =  7.1;
aisle_center_y = 0.10;

bay_length = 4.30;
bay_width  = 3.40;
bay_angle  = 15*pi/180;
bay_center_x = 0.0;
bay_center_y = 2.70;

%% Rear-axle start and goal poses
start_pose = [-5.0, 0.0, pi];

% The bay centre is a BODY-centre position, not a rear-axle position.
body_center_from_rear_axle = (veh(3) + veh(5) - veh(6))/2;
goal_pose = [ ...
    bay_center_x - body_center_from_rear_axle*cos(bay_angle), ...
    bay_center_y - body_center_from_rear_axle*sin(bay_angle), ...
    bay_angle];

%% Occupancy grid
% Stateless: each call reflects the dimensions above, without a cached map.
[IX,IY] = meshgrid(0:W-1,0:H-1);
X = origin_x + IX*res;
Y = origin_y + IY*res;

% Avoid asymmetric inclusion of boundary points due to floating-point error.
tol = 1e-9;
% These walls coincide with cell edges. Include only complete free cells.
% The start is 0.10 m below the aisle centreline.
aisle = X >= aisle_x_min+res/2-tol & X <= aisle_x_max-res/2+tol & ...
        abs(Y-aisle_center_y) <= aisle_width/2-res/2+tol;

% Coordinates along/across the angled bay.
dx = X-bay_center_x;
dy = Y-bay_center_y;
along  =  cos(bay_angle)*dx + sin(bay_angle)*dy;
across = -sin(bay_angle)*dx + cos(bay_angle)*dy;
bay = abs(along) <= bay_length/2+tol & ...
      abs(across) <= bay_width/2+tol;

% Free space is the union of the aisle and bay. Everything else is occupied.
% No obstacle inflation is added here. The planner handles its ego margin.
occupied = ~(aisle | bay);

%% Existing OccupancyGrid bus format
costmap.info.resolution = res;
costmap.info.width  = uint32(W);
costmap.info.height = uint32(H);
costmap.info.origin.position.x = origin_x;
costmap.info.origin.position.y = origin_y;
costmap.info.origin.position.z = 0;
costmap.info.origin.orientation.x = 0;
costmap.info.origin.orientation.y = 0;
costmap.info.origin.orientation.z = 0;
costmap.info.origin.orientation.w = 1;
costmap.data = int8(occupied).*int8(100);
end

== matlab function ATOM_parking_chain/Parking Scenario1/Costmap generation: obstacle2/MATLAB Function ==
  settings: updateMethod=DISCRETE
  data: costmap output Bus: OccupancyGridBus; start_pose output; goal_pose output; veh input
function [costmap, start_pose, goal_pose] = costmapUndergroundParking(veh)
%COSTMAPUNDERGROUNDPARKING  Realistic reverse parking in a double-row garage.
% The target is the empty bay at x = 0 in the upper row. Parked vehicles
% surround it, an opposing row limits the aisle, and a structural column is
% located beside the entrance. Poses refer to the rear-axle centre.

%% Fixed OccupancyGrid dimensions used by the current model
res = 0.20;
W = 234;
H = 234;
origin_x = -(W/2)*res;
origin_y = -(H/2)*res;
[IX,IY] = meshgrid(0:W-1,0:H-1);
X = origin_x + IX*res;
Y = origin_y + IY*res;

%% Garage geometry [m]
aisle_width = 6.50;       % clear nominal two-way manoeuvring aisle
parking_depth = 5.20;
bay_pitch = 3.20;         % centre-to-centre bay spacing
parked_length = 4.60;     % physical parked vehicle, no inflation here
parked_width = 2.00;
pillar_size = 0.40;

garage_x_min = -11.0;
garage_x_max =  11.0;
garage_y_min = -(aisle_width/2 + parking_depth);
garage_y_max =  (aisle_width/2 + parking_depth);

% Start occupied and carve out the garage floor.
occupied = true(H,W);
garage_floor = X >= garage_x_min & X <= garage_x_max & ...
               Y >= garage_y_min & Y <= garage_y_max;
occupied(garage_floor) = false;

%% Parked vehicles
row_y = aisle_width/2 + parking_depth/2;
bay_x = (-3:3)*bay_pitch;

for k = 1:numel(bay_x)
    % Upper row: leave the centre bay empty.
    if k ~= 4
        top_car = abs(X-bay_x(k)) <= parked_width/2 & ...
                  abs(Y-row_y) <= parked_length/2;
        occupied(top_car) = true;
    end

    % Opposing row: all bays occupied.
    bottom_car = abs(X-bay_x(k)) <= parked_width/2 & ...
                 abs(Y+row_y) <= parked_length/2;
    occupied(bottom_car) = true;
end

%% Structural column beside the target bay entrance
pillar_x = bay_pitch/2;
pillar_y = aisle_width/2 + pillar_size/2 + 0.10;
pillar = abs(X-pillar_x) <= pillar_size/2 & ...
         abs(Y-pillar_y) <= pillar_size/2;
occupied(pillar) = true;

%% Parking task
% The vehicle begins beside the target bay, as it would after approaching
% through the aisle, and reverses into the upper-row space.
start_pose = [-5.0, 0.0, pi/2];
goal_pose = [0.0, row_y, -pi/2];

%% Existing OccupancyGrid bus format
costmap.info.resolution = res;
costmap.info.width = uint32(W);
costmap.info.height = uint32(H);
costmap.info.origin.position.x = origin_x;
costmap.info.origin.position.y = origin_y;
costmap.info.origin.position.z = 0;
costmap.info.origin.orientation.x = 0;
costmap.info.origin.orientation.y = 0;
costmap.info.origin.orientation.z = 0;
costmap.info.origin.orientation.w = 1;
costmap.data = int8(occupied).*int8(100);

% veh is intentionally kept as the input because the surrounding subsystem
% already supplies the 29-element vehicle vector and all costmap blocks use
% the same interface. Geometry above represents other parked vehicles.
if numel(veh) < 8
    error('costmapUndergroundParking:VehSize', ...
        'veh must be the complete vehicle-parameter vector.');
end
end

== matlab function ATOM_parking_chain/Parking Scenario1/Costmap generation: parking scenario beside a lane/MATLAB Function ==
  settings: updateMethod=DISCRETE
  data: veh input; costmap output Bus: OccupancyGridBus; start_pose output; goal_pose output
function [costmap, start_pose, goal_pose] = costmapDoubleRowLot(veh)
%COSTMAPDOUBLEROWLOT  Two rows of bays with a realistic aisle between them.
%
% Harder than the single-row lot: the car must enter the bay from an 8.6 m
% aisle with a 5.47 m turning radius, so it cannot swing in with one arc.
%
% Reproduces autoware_costmap_generator geometry:
%   grid_resolution 0.3, grid_length_x/y 70.0, expand_polygon_size 0.5

persistent occ

res = 0.3;   W = 234;   H = 234;
origin_x = -(W/2)*res;
origin_y = -(H/2)*res;

bay_x   = (-2:2)*3.6;          % 5 bays per row, 3.6 m pitch
row_y   = 6.0;                 % rows at y = +6 and y = -6  -> 8.6 m aisle
free_bay = 3;                  % the empty one, top row (x = 0)

if isempty(occ)
    [IX, IY] = meshgrid(0:W-1, 0:H-1);
    X = origin_x + IX*res;
    Y = origin_y + IY*res;

    % the lot, carved out of the wall
    lot_x = [-12  12  12 -12];
    lot_y = [ -9  -9   9   9];
    occ = ones(H,W);
    occ(inpolygon(X, Y, lot_x, lot_y)) = 0;

    car_len = veh(5) + veh(3) + veh(6);
    car_wid = veh(4) + veh(7) + veh(8);
    expand  = 0.5;
    L = car_len + expand;
    D = car_wid + expand;

    for k = 1:5
        % top row, one bay left empty
        if k ~= free_bay
            qx = [ D/2 -D/2 -D/2  D/2] + bay_x(k);
            qy = [ L/2  L/2 -L/2 -L/2] + row_y;
            occ(inpolygon(X, Y, qx, qy)) = 1;
        end
        % bottom row, fully occupied
        qx = [ D/2 -D/2 -D/2  D/2] + bay_x(k);
        qy = [ L/2  L/2 -L/2 -L/2] - row_y;
        occ(inpolygon(X, Y, qx, qy)) = 1;
    end
end

% --- the poses that belong to this scene ---------------------------------
start_pose = [-8, 0, 0];                    % in the aisle, heading east
goal_pose  = [ 0, row_y , pi/2 + pi];       % nose-in, top row, x = 0

costmap.info.resolution           = res;
costmap.info.width                = uint32(W);
costmap.info.height               = uint32(H);
costmap.info.origin.position.x    = origin_x;
costmap.info.origin.position.y    = origin_y;
costmap.info.origin.position.z    = 0;
costmap.info.origin.orientation.x = 0;
costmap.info.origin.orientation.y = 0;
costmap.info.origin.orientation.z = 0;
costmap.info.origin.orientation.w = 1;
costmap.data                      = int8(occ*100);
end

== matlab function ATOM_parking_chain/Parking Scenario1/Costmap generation: perpendicular lot/Perpendicular Parking ==
  settings: updateMethod=DISCRETE
  data: veh input; costmap output Bus: OccupancyGridBus; start_pose output; goal_pose output
function [costmap, start_pose, goal_pose] = costmapPerpendicularLot(veh)
%COSTMAPPERPENDICULARLOT  Single row of 7 bays, one left empty at x = 0.
%
% Reproduces autoware_costmap_generator geometry:
%   grid_resolution 0.3, grid_length_x/y 70.0, expand_polygon_size 0.5
% The primitives layer is INVERTED: background occupied, lot carved out.

persistent occ

res = 0.3;   W = 234;   H = 234;
origin_x = -(W/2)*res;
origin_y = -(H/2)*res;

bay_x     = (-3:3)*3.6;      % 7 bays, 3.6 m pitch
bay_y     = 8.75;
empty_bay = 4;               % x = 0

if isempty(occ)
    [IX, IY] = meshgrid(0:W-1, 0:H-1);
    X = origin_x + IX*res;
    Y = origin_y + IY*res;

    lot_x = [-15  15  15 -15];
    lot_y = [-12 -12  12  12];
    occ = ones(H,W);
    occ(inpolygon(X, Y, lot_x, lot_y)) = 0;

    car_len = veh(5) + veh(3) + veh(6);
    car_wid = veh(4) + veh(7) + veh(8);
    expand  = 0.5;
    L = car_len + expand;
    D = car_wid + expand;

    for k = 1:7
        if k ~= empty_bay
            qx = [ D/2 -D/2 -D/2  D/2] + bay_x(k);
            qy = [ L/2  L/2 -L/2 -L/2] + bay_y;
            occ(inpolygon(X, Y, qx, qy)) = 1;
        end
    end
end

start_pose = [0, 0,    0];
goal_pose  = [0, 7.75, pi/2];

costmap.info.resolution           = res;
costmap.info.width                = uint32(W);
costmap.info.height               = uint32(H);
costmap.info.origin.position.x    = origin_x;
costmap.info.origin.position.y    = origin_y;
costmap.info.origin.position.z    = 0;
costmap.info.origin.orientation.x = 0;
costmap.info.origin.orientation.y = 0;
costmap.info.origin.orientation.z = 0;
costmap.info.origin.orientation.w = 1;
costmap.data                      = int8(occ*100);
end

== matlab function ATOM_parking_chain/Parking Scenario1/MATLAB Function ==
  data: segment_done input; segment_request output; segment_count input; maneuver_complete output
function [segment_request, maneuver_complete] = ...
    segmentManager(segment_done, segment_count)
%SEGMENTMANAGER
% Advance exactly once when the current segment is completed.

persistent active_segment previous_done complete_latched

if isempty(active_segment)
    active_segment  = 1.0;
    previous_done   = false;
    complete_latched = false;
end

% Convert the inputs into known scalar types.
done_now = logical(segment_done);
count = max(0.0, floor(double(segment_count)));

% Protect against an active index larger than the available count.
if count > 0 && active_segment > count
    active_segment = count;
end

% Detect only the transition from not-done to done.
done_rising_edge = done_now && ~previous_done;

if done_rising_edge && count > 0

    if active_segment < count

        % Another segment exists.
        active_segment = active_segment + 1.0;

    else

        % The final segment has been completed.
        complete_latched = true;

    end
end

previous_done = done_now;

segment_request  = active_segment;
maneuver_complete = complete_latched;
end
